simulink model "Rail_RegenerativeBraking_TianjinMetro_MotorSelection_v1"  (R2025a)
settings: Solver=ode23tb  StartTime=0.0  StopTime=SCv1.scenario.stop_time  FixedStep=Ts  MaxStep=Ts  RelTol=1e-4  EnableMultiTasking=on
PreLoadFcn:
  | SCv1_root=fileparts(fileparts(get_param(bdroot,'FileName'))); run(fullfile(SCv1_root,'config','SC_v1_parameters.m')); clear SCv1_root;
model workspace (MAT data in the model file):
  MotorCandidateIDs = {'A', 'B', 'C', 'D'}
  MotorSurrogateStatement = 'parameterized surrogate traction motor model based on published nameplate data'
  TianjinMetroBaseline.city = 'Tianjin'
  TianjinMetroBaseline.train_type = 'metro_B'
  TianjinMetroBaseline.cars = 6
  TianjinMetroBaseline.max_operation_speed_kmh = 80
  TianjinMetroBaseline.design_speed_kmh = 90
  TianjinMetroBaseline.wheel_radius_m = 0.42
  TianjinMetroBaseline.motor_count = 16
  TianjinMetroBaseline.aw2_mass_kg = 292080
  TianjinMetroBaseline.aw3_mass_kg = 316800
undefined symbols (not defined in the file): DiscIntNeverNeededParam, flux, Ld, Lq, Pn, SCv1, Ts
libraries: spsSeriesRLCBranchLib x5, spsControlledCurrentSourceLib x3, spsCurrentMeasurementLib x3, spsVoltageMeasurementLib x3, powerlib_extras x2, spsDCVoltageSourceLib x1, spsDiodeLib x1, spsPermanentMagnetSynchronousMachineLib x1, simulink x1, spsUniversalBridgeLib x1, sps_lib x1
(part 1 of 2)
Description:
  | Tianjin Metro B-type 6-car motor selection derivative. Candidate dynamics are supplied by parameterized published-nameplate FMUs.
settings Model: Creator=SUN  LastModifiedBy=AUSA
settings SolverCC: ZeroCrossControl=DisableAll  AlgebraicLoopSolver=TrustRegion
settings DataIOCC: LimitDataPoints=on  SaveFormat=Array  SignalLoggingSaveFormat=ModelDataLogs
settings OptimizationCC: ExpressionDepthLimit=2147483647.0  InitFltsAndDblsToZero=on  LifeSpan=inf
settings DebuggingCC: UnderspecifiedInitializationDetection=Classic  MergeDetectMultiDrivingBlocksExec=none  SolverPrmCheckMsg=warning  FcnCallInpInsideContextMsg=warning  UnconnectedInputMsg=warning  UnconnectedOutputMsg=warning  UnconnectedLineMsg=warning  StateNameClashWarn=warning  SFUnexpectedBacktrackingDiag=warning  SFNoUnconditionalDefaultTransitionDiag=warning  ArithmeticOperatorsInVariantConditions=warning
settings HardwareCC: ProdBitPerPointer=32.0  ProdBitPerSizeT=32.0  ProdBitPerPtrDiffT=32.0  ProdLargestAtomicFloat=None  ProdIntDivRoundTo=Undefined  ProdEndianess=Unspecified  ProdWordSize=32.0  ProdHWDeviceType=32-bit Generic
settings ModelReferenceCC: EnableRefExpFcnMdlSchedulingChecks=on  PropagateSignalLabelsOutOfModel=off
settings SFSimCC: SimUseLocalCustomCode=off  CustomCodeUndefinedFunction=UseInterfaceOnly
settings RTWCC: RTWUseLocalCustomCode=off  GPUComputeCapability=3.5
settings CodeAppCC: StateflowObjectComments=on
settings GRTTargetCC: TargetLangStandard=C89/C90 (ANSI)  CombineOutputUpdateFcns=off  GRTInterface=on
settings ConfigComp: CovMetricSettings=dw  CovSaveCumulativeToWorkspaceVar=on  CovSaveSingleToWorkspaceVar=on  CovExternalEMLEnable=off  CovSFcnEnable=off
settings SimscapeCC: SimscapeNormalizeSystem=off

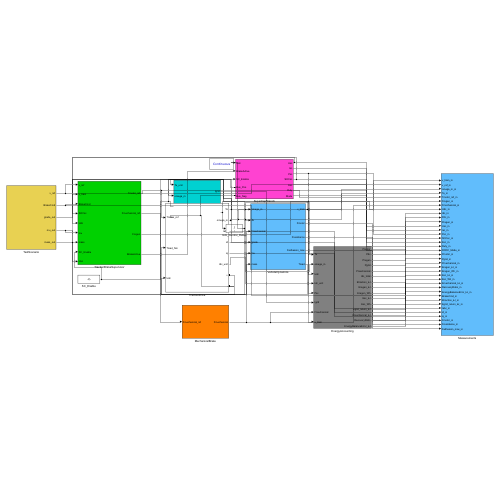
[thumbnail: Simulink's stored preview of the top-level diagram]
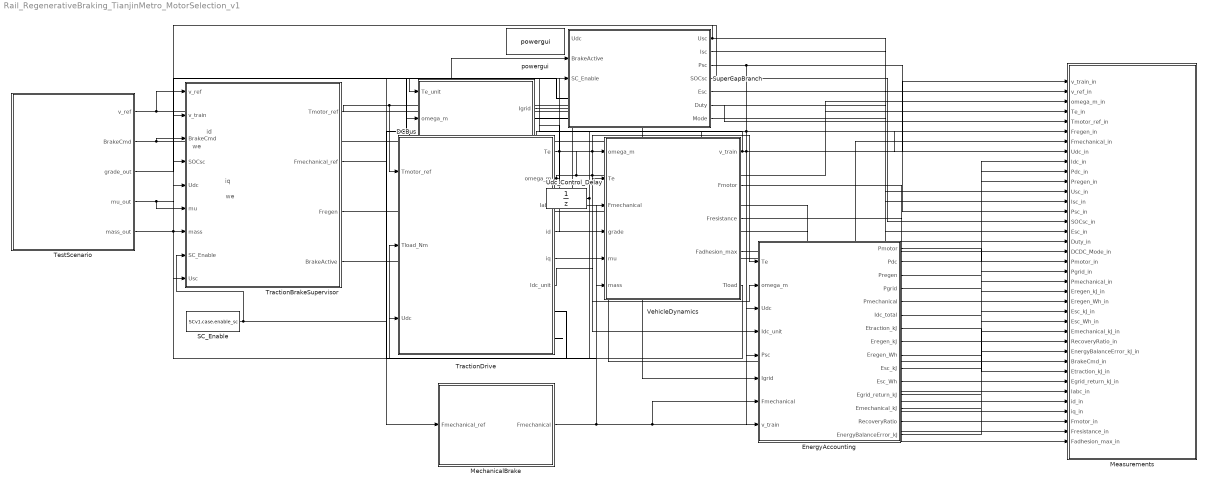
== system Rail_RegenerativeBraking_TianjinMetro_MotorSelection_v1 ==
  note: iq
  note: we
  note: we
  note: id
  DCBus : Subsystem
  EnergyAccounting : Subsystem
  Measurements : Subsystem
  MechanicalBrake : Subsystem
  SC_Enable : Constant  Value=SCv1.case.enable_sc
  SuperCapBranch : Subsystem
  TestScenario : Subsystem
  TractionBrakeSupervisor : Subsystem
  TractionDrive : Subsystem
  Udc_Control_Delay : UnitDelay  InitialCondition=SCv1.dc.Udc_initial  SampleTime=Ts  HasFrameUpgradeWarning=on
  VehicleDynamics : Subsystem
  powergui : sps_lib/powergui  SimulationMode=Continuous  SampleTime=Ts  frequency=60  Iterations=50  frequencyindice=0  Pbase=100e6  ErrMax=1e-4  UnitsV=kV  UnitsW=MW  buscounter=0  FunctionMessages=off  echomessages=off  EnableUseOfTLC=off  CurrentSourceSwitches=on  DisableSnubberDevices=off  DisableRonSwitches=off  DisableVfSwitches=off  DisplayEquations=off  AutomaticDiscreteSolvers=off  SolverType=Tustin/Backward Euler (TBE)  Interpol=off  ExternalGateDelay=off  methode=off  Ts=0  x0status=blocks  SPID=off  SwTol=0  HookPort=off  NonlinearTolerance=1e-4  nMaxIteration=100  ContinueOnMaxIteration=off  RestoreLinks=warning  ResistiveCurrentMeasurement=off  Frange=[0:2:500]  Ylog=off  Xlog=on  ShowGrid=off  save=off  variable=ZData  structure=0  ZoomFFT=on  StartTime=0.0  cycles=1  DisplayStyle=1  fundamental=60  FreqAxis=off  MaxFrequency=1000  frequencyindicesteady=1  RmsSteady=1  display=off
  wires:
  TestScenario/1(v_ref) -> TractionBrakeSupervisor/1(v_ref), Measurements/2(v_ref_in)
  VehicleDynamics/1(v_train) -> EnergyAccounting/8(v_train), Measurements/1(v_train_in), TractionBrakeSupervisor/2(v_train)
  TestScenario/2(BrakeCmd) -> TractionBrakeSupervisor/3(BrakeCmd), Measurements/29(BrakeCmd_in)
  SuperCapBranch/4(SOCsc) -> TractionBrakeSupervisor/4(SOCsc), Measurements/15(SOCsc_in)
  DCBus/2(Udc) -> EnergyAccounting/3(Udc), Measurements/8(Udc_in), Udc_Control_Delay/1
  TestScenario/4(mu_out) -> TractionBrakeSupervisor/6(mu), VehicleDynamics/5(mu)
  TestScenario/5(mass_out) -> TractionBrakeSupervisor/7(mass), VehicleDynamics/6(mass)
  SC_Enable/1 -> TractionBrakeSupervisor/8(SC_Enable), SuperCapBranch/3(SC_Enable)
  SuperCapBranch/1(Usc) -> TractionBrakeSupervisor/9(Usc), Measurements/12(Usc_in)
  TractionBrakeSupervisor/1(Tmotor_ref) -> TractionDrive/1(Tmotor_ref), Measurements/5(Tmotor_ref_in)
  TractionBrakeSupervisor/2(Fmechanical_ref) -> MechanicalBrake/1(Fmechanical_ref)
  MechanicalBrake/1(Fmechanical) -> EnergyAccounting/7(Fmechanical), Measurements/7(Fmechanical_in), VehicleDynamics/3(Fmechanical)
  TractionDrive/2(omega_m) -> EnergyAccounting/2(omega_m), Measurements/3(omega_m_in), VehicleDynamics/1(omega_m), DCBus/2(omega_m)
  TractionDrive/1(Te) -> VehicleDynamics/2(Te), EnergyAccounting/1(Te), Measurements/4(Te_in), DCBus/1(Te_unit)
  TestScenario/3(grade_out) -> VehicleDynamics/4(grade)
  VehicleDynamics/5(Tload) -> TractionDrive/2(Tload_Nm)
  TractionDrive/6(Idc_unit) -> EnergyAccounting/4(Idc_unit)
  TractionBrakeSupervisor/4(BrakeActive) -> SuperCapBranch/2(BrakeActive)
  SuperCapBranch/3(Psc) -> EnergyAccounting/5(Psc), Measurements/14(Psc_in)
  DCBus/1(Igrid) -> EnergyAccounting/6(Igrid)
  TractionBrakeSupervisor/3(Fregen) -> Measurements/6(Fregen_in)
  EnergyAccounting/6(Idc_total) -> Measurements/9(Idc_in)
  EnergyAccounting/2(Pdc) -> Measurements/10(Pdc_in)
  EnergyAccounting/3(Pregen) -> Measurements/11(Pregen_in)
  SuperCapBranch/2(Isc) -> Measurements/13(Isc_in)
  SuperCapBranch/5(Esc) -> Measurements/16(Esc_in)
  SuperCapBranch/6(Duty) -> Measurements/17(Duty_in)
  SuperCapBranch/7(Mode) -> Measurements/18(DCDC_Mode_in)
  EnergyAccounting/1(Pmotor) -> Measurements/19(Pmotor_in)
  EnergyAccounting/4(Pgrid) -> Measurements/20(Pgrid_in)
  EnergyAccounting/5(Pmechanical) -> Measurements/21(Pmechanical_in)
  EnergyAccounting/8(Eregen_kJ) -> Measurements/22(Eregen_kJ_in)
  EnergyAccounting/9(Eregen_Wh) -> Measurements/23(Eregen_Wh_in)
  EnergyAccounting/10(Esc_kJ) -> Measurements/24(Esc_kJ_in)
  EnergyAccounting/11(Esc_Wh) -> Measurements/25(Esc_Wh_in)
  EnergyAccounting/13(Emechanical_kJ) -> Measurements/26(Emechanical_kJ_in)
  EnergyAccounting/14(RecoveryRatio) -> Measurements/27(RecoveryRatio_in)
  EnergyAccounting/15(EnergyBalanceError_kJ) -> Measurements/28(EnergyBalanceError_kJ_in)
  Udc_Control_Delay/1 -> TractionDrive/3(Udc), TractionBrakeSupervisor/5(Udc), SuperCapBranch/1(Udc)
  EnergyAccounting/7(Etraction_kJ) -> Measurements/30(Etraction_kJ_in)
  EnergyAccounting/12(Egrid_return_kJ) -> Measurements/31(Egrid_return_kJ_in)
  TractionDrive/3(Iabc) -> Measurements/32(Iabc_in)
  TractionDrive/4(id) -> Measurements/33(id_in)
  TractionDrive/5(iq) -> Measurements/34(iq_in)
  VehicleDynamics/2(Fmotor) -> Measurements/35(Fmotor_in)
  VehicleDynamics/3(Fresistance) -> Measurements/36(Fresistance_in)
  VehicleDynamics/4(Fadhesion_max) -> Measurements/37(Fadhesion_max_in)
  connections:
  TractionDrive/RConn1 -- DCBus/LConn1 -- SuperCapBranch/LConn1
  TractionDrive/RConn2 -- DCBus/LConn2 -- SuperCapBranch/LConn2

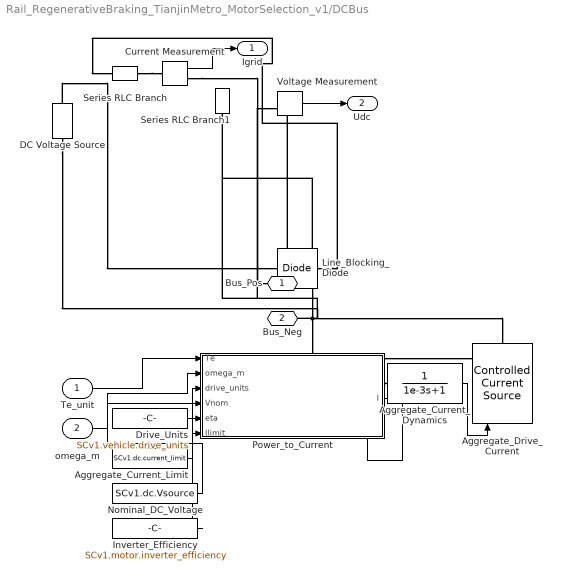
== system Rail_RegenerativeBraking_TianjinMetro_MotorSelection_v1/DCBus ==
  Te_unit : Inport
  omega_m : Inport  Port=2
  Aggregate_Current_Dynamics : TransferFcn  Numerator=1  Denominator=[1e-3 1]
  Aggregate_Current_Limit : Constant  Value=SCv1.dc.current_limit
  Aggregate_Drive_Current : spsControlledCurrentSourceLib/Controlled Current Source  Initialize=off  Source_Type=AC  Amplitude=0  Phase=0  Frequency=0  Measurements=None
  Current Measurement : spsCurrentMeasurementLib/Current Measurement  PhasorSimulation=off  OutputType=Complex  PSBequivalent=0
  DC Voltage Source : spsDCVoltageSourceLib/DC Voltage Source  Amplitude=SCv1.dc.Vsource  Measurements=None
  Drive_Units : Constant  Value=SCv1.vehicle.drive_units
  Inverter_Efficiency : Constant  Value=SCv1.motor.inverter_efficiency
  Line_Blocking_Diode : spsDiodeLib/Diode  Ron=1e-3  Lon=0  Vf=0.8  IC=0  UseSnubber=1  Rs=1e5  Cs=inf  Measurements=off
  Nominal_DC_Voltage : Constant  Value=SCv1.dc.Vsource
  Power_to_Current : MATLAB Function  TreatAsAtomicUnit=on
  Series RLC Branch : spsSeriesRLCBranchLib/Series RLC Branch  LConnTagsString=__new0  RConnTagsString=__new0  BranchType=RL  Resistance=SCv1.dc.line_R  Inductance=SCv1.dc.line_L  SetiL0=off  InitialCurrent=0  Capacitance=1e-6  Setx0=off  InitialVoltage=0  Measurements=None
  Series RLC Branch1 : spsSeriesRLCBranchLib/Series RLC Branch  LConnTagsString=__new0  RConnTagsString=__new0  BranchType=C  Resistance=25  Inductance=1e-3  SetiL0=off  InitialCurrent=0  Capacitance=SCv1.dc.Cdc  Setx0=on  InitialVoltage=SCv1.dc.Udc_initial  Measurements=None
  Voltage Measurement : spsVoltageMeasurementLib/Voltage Measurement  PhasorSimulation=off  OutputType=Complex  PSBequivalent=0
  Bus_Pos : PMIOPort  Side=Left
  Bus_Neg : PMIOPort  Port=2  Side=Left
  Igrid : Outport
  Udc : Outport  Port=2
  wires:
  Current Measurement/1 -> Igrid/1
  Voltage Measurement/1 -> Udc/1
  Power_to_Current/1(I) -> Aggregate_Current_Dynamics/1
  Aggregate_Current_Dynamics/1 -> Aggregate_Drive_Current/1
  Te_unit/1 -> Power_to_Current/1(Te)
  omega_m/1 -> Power_to_Current/2(omega_m)
  Drive_Units/1 -> Power_to_Current/3(drive_units)
  Nominal_DC_Voltage/1 -> Power_to_Current/4(Vnom)
  Inverter_Efficiency/1 -> Power_to_Current/5(eta)
  Aggregate_Current_Limit/1 -> Power_to_Current/6(Ilimit)
  connections:
  DC Voltage Source/RConn1 -- Line_Blocking_Diode/LConn1
  Line_Blocking_Diode/RConn1 -- Series RLC Branch/LConn1
  Series RLC Branch/RConn1 -- Current Measurement/LConn1
  Current Measurement/RConn1 -- Series RLC Branch1/LConn1 -- Voltage Measurement/LConn1 -- Bus_Pos/RConn1 -- Aggregate_Drive_Current/LConn1
  DC Voltage Source/LConn1 -- Series RLC Branch1/RConn1 -- Voltage Measurement/LConn2 -- Bus_Neg/RConn1 -- Aggregate_Drive_Current/RConn1

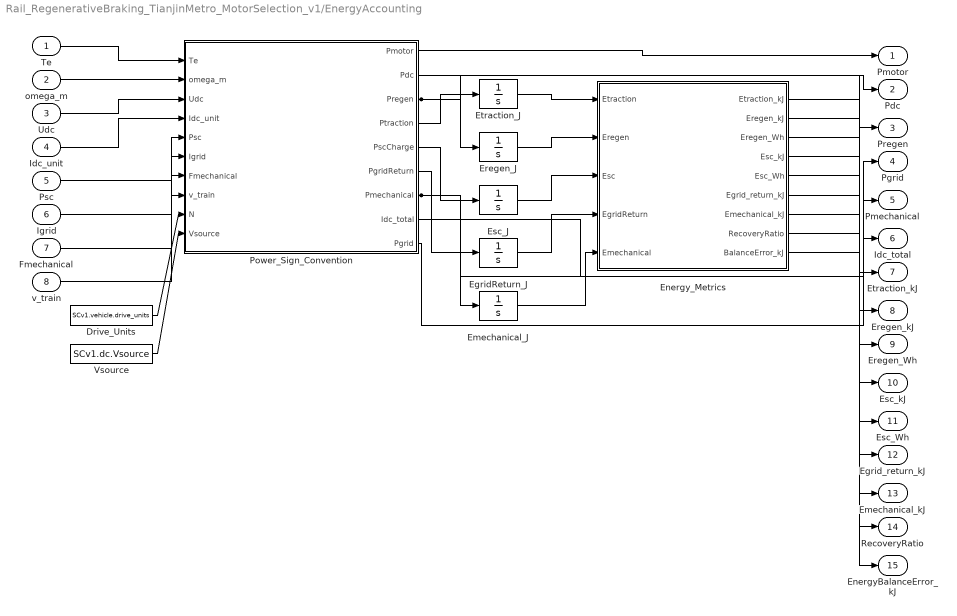
== system Rail_RegenerativeBraking_TianjinMetro_MotorSelection_v1/EnergyAccounting ==
  Te : Inport
  omega_m : Inport  Port=2
  Udc : Inport  Port=3
  Idc_unit : Inport  Port=4
  Psc : Inport  Port=5
  Igrid : Inport  Port=6
  Fmechanical : Inport  Port=7
  v_train : Inport  Port=8
  Drive_Units : Constant  Value=SCv1.vehicle.drive_units
  EgridReturn_J : Integrator
  Emechanical_J : Integrator
  Energy_Metrics : MATLAB Function  TreatAsAtomicUnit=on
  Eregen_J : Integrator
  Esc_J : Integrator
  Etraction_J : Integrator
  Power_Sign_Convention : MATLAB Function  TreatAsAtomicUnit=on
  Vsource : Constant  Value=SCv1.dc.Vsource
  Pmotor : Outport
  Pdc : Outport  Port=2
  Pregen : Outport  Port=3
  Pgrid : Outport  Port=4
  Pmechanical : Outport  Port=5
  Idc_total : Outport  Port=6
  Etraction_kJ : Outport  Port=7
  Eregen_kJ : Outport  Port=8
  Eregen_Wh : Outport  Port=9
  Esc_kJ : Outport  Port=10
  Esc_Wh : Outport  Port=11
  Egrid_return_kJ : Outport  Port=12
  Emechanical_kJ : Outport  Port=13
  RecoveryRatio : Outport  Port=14
  EnergyBalanceError_kJ : Outport  Port=15
  wires:
  Te/1 -> Power_Sign_Convention/1(Te)
  omega_m/1 -> Power_Sign_Convention/2(omega_m)
  Udc/1 -> Power_Sign_Convention/3(Udc)
  Idc_unit/1 -> Power_Sign_Convention/4(Idc_unit)
  Psc/1 -> Power_Sign_Convention/5(Psc)
  Igrid/1 -> Power_Sign_Convention/6(Igrid)
  Fmechanical/1 -> Power_Sign_Convention/7(Fmechanical)
  v_train/1 -> Power_Sign_Convention/8(v_train)
  Drive_Units/1 -> Power_Sign_Convention/9(N)
  Vsource/1 -> Power_Sign_Convention/10(Vsource)
  Power_Sign_Convention/4(Ptraction) -> Etraction_J/1
  Power_Sign_Convention/3(Pregen) -> Eregen_J/1, Pregen/1
  Power_Sign_Convention/5(PscCharge) -> Esc_J/1
  Power_Sign_Convention/6(PgridReturn) -> EgridReturn_J/1
  Power_Sign_Convention/7(Pmechanical) -> Emechanical_J/1, Pmechanical/1
  Etraction_J/1 -> Energy_Metrics/1(Etraction)
  Eregen_J/1 -> Energy_Metrics/2(Eregen)
  Esc_J/1 -> Energy_Metrics/3(Esc)
  EgridReturn_J/1 -> Energy_Metrics/4(EgridReturn)
  Emechanical_J/1 -> Energy_Metrics/5(Emechanical)
  Power_Sign_Convention/1(Pmotor) -> Pmotor/1
  Power_Sign_Convention/2(Pdc) -> Pdc/1
  Power_Sign_Convention/9(Pgrid) -> Pgrid/1
  Power_Sign_Convention/8(Idc_total) -> Idc_total/1
  Energy_Metrics/1(Etraction_kJ) -> Etraction_kJ/1
  Energy_Metrics/2(Eregen_kJ) -> Eregen_kJ/1
  Energy_Metrics/3(Eregen_Wh) -> Eregen_Wh/1
  Energy_Metrics/4(Esc_kJ) -> Esc_kJ/1
  Energy_Metrics/5(Esc_Wh) -> Esc_Wh/1
  Energy_Metrics/6(Egrid_return_kJ) -> Egrid_return_kJ/1
  Energy_Metrics/7(Emechanical_kJ) -> Emechanical_kJ/1
  Energy_Metrics/8(RecoveryRatio) -> RecoveryRatio/1
  Energy_Metrics/9(BalanceError_kJ) -> EnergyBalanceError_kJ/1

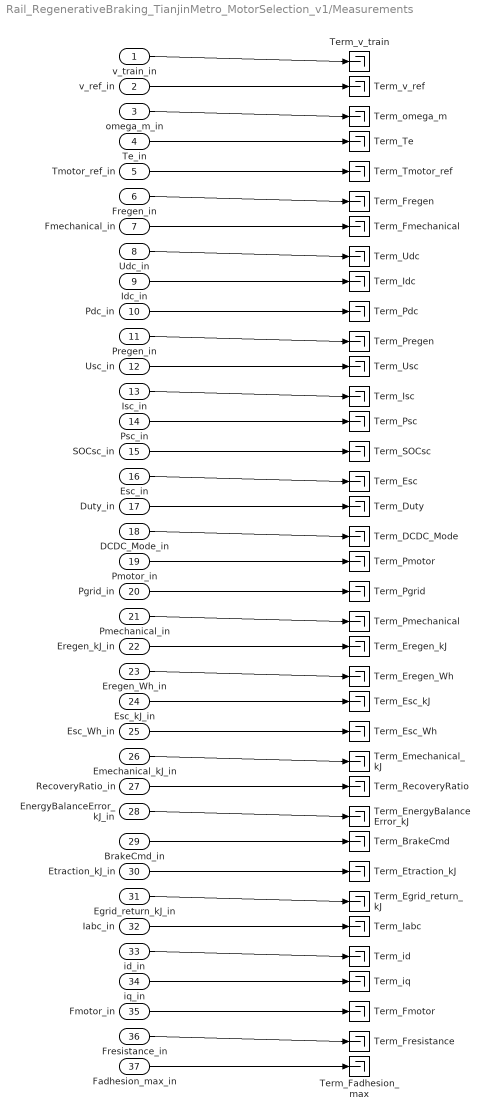
== system Rail_RegenerativeBraking_TianjinMetro_MotorSelection_v1/Measurements ==
  v_train_in : Inport
  v_ref_in : Inport  Port=2
  omega_m_in : Inport  Port=3
  Te_in : Inport  Port=4
  Tmotor_ref_in : Inport  Port=5
  Fregen_in : Inport  Port=6
  Fmechanical_in : Inport  Port=7
  Udc_in : Inport  Port=8
  Idc_in : Inport  Port=9
  Pdc_in : Inport  Port=10
  Pregen_in : Inport  Port=11
  Usc_in : Inport  Port=12
  Isc_in : Inport  Port=13
  Psc_in : Inport  Port=14
  SOCsc_in : Inport  Port=15
  Esc_in : Inport  Port=16
  Duty_in : Inport  Port=17
  DCDC_Mode_in : Inport  Port=18
  Pmotor_in : Inport  Port=19
  Pgrid_in : Inport  Port=20
  Pmechanical_in : Inport  Port=21
  Eregen_kJ_in : Inport  Port=22
  Eregen_Wh_in : Inport  Port=23
  Esc_kJ_in : Inport  Port=24
  Esc_Wh_in : Inport  Port=25
  Emechanical_kJ_in : Inport  Port=26
  RecoveryRatio_in : Inport  Port=27
  EnergyBalanceError_kJ_in : Inport  Port=28
  BrakeCmd_in : Inport  Port=29
  Etraction_kJ_in : Inport  Port=30
  Egrid_return_kJ_in : Inport  Port=31
  Iabc_in : Inport  Port=32
  id_in : Inport  Port=33
  iq_in : Inport  Port=34
  Fmotor_in : Inport  Port=35
  Fresistance_in : Inport  Port=36
  Fadhesion_max_in : Inport  Port=37
  Term_BrakeCmd : Terminator
  Term_DCDC_Mode : Terminator
  Term_Duty : Terminator
  Term_Egrid_return_kJ : Terminator
  Term_Emechanical_kJ : Terminator
  Term_EnergyBalanceError_kJ : Terminator
  Term_Eregen_Wh : Terminator
  Term_Eregen_kJ : Terminator
  Term_Esc : Terminator
  Term_Esc_Wh : Terminator
  Term_Esc_kJ : Terminator
  Term_Etraction_kJ : Terminator
  Term_Fadhesion_max : Terminator
  Term_Fmechanical : Terminator
  Term_Fmotor : Terminator
  Term_Fregen : Terminator
  Term_Fresistance : Terminator
  Term_Iabc : Terminator
  Term_Idc : Terminator
  Term_Isc : Terminator
  Term_Pdc : Terminator
  Term_Pgrid : Terminator
  Term_Pmechanical : Terminator
  Term_Pmotor : Terminator
  Term_Pregen : Terminator
  Term_Psc : Terminator
  Term_RecoveryRatio : Terminator
  Term_SOCsc : Terminator
  Term_Te : Terminator
  Term_Tmotor_ref : Terminator
  Term_Udc : Terminator
  Term_Usc : Terminator
  Term_id : Terminator
  Term_iq : Terminator
  Term_omega_m : Terminator
  Term_v_ref : Terminator
  Term_v_train : Terminator
  wires:
  v_train_in/1 -> Term_v_train/1
  v_ref_in/1 -> Term_v_ref/1
  omega_m_in/1 -> Term_omega_m/1
  Te_in/1 -> Term_Te/1
  Tmotor_ref_in/1 -> Term_Tmotor_ref/1
  Fregen_in/1 -> Term_Fregen/1
  Fmechanical_in/1 -> Term_Fmechanical/1
  Udc_in/1 -> Term_Udc/1
  Idc_in/1 -> Term_Idc/1
  Pdc_in/1 -> Term_Pdc/1
  Pregen_in/1 -> Term_Pregen/1
  Usc_in/1 -> Term_Usc/1
  Isc_in/1 -> Term_Isc/1
  Psc_in/1 -> Term_Psc/1
  SOCsc_in/1 -> Term_SOCsc/1
  Esc_in/1 -> Term_Esc/1
  Duty_in/1 -> Term_Duty/1
  DCDC_Mode_in/1 -> Term_DCDC_Mode/1
  Pmotor_in/1 -> Term_Pmotor/1
  Pgrid_in/1 -> Term_Pgrid/1
  Pmechanical_in/1 -> Term_Pmechanical/1
  Eregen_kJ_in/1 -> Term_Eregen_kJ/1
  Eregen_Wh_in/1 -> Term_Eregen_Wh/1
  Esc_kJ_in/1 -> Term_Esc_kJ/1
  Esc_Wh_in/1 -> Term_Esc_Wh/1
  Emechanical_kJ_in/1 -> Term_Emechanical_kJ/1
  RecoveryRatio_in/1 -> Term_RecoveryRatio/1
  EnergyBalanceError_kJ_in/1 -> Term_EnergyBalanceError_kJ/1
  BrakeCmd_in/1 -> Term_BrakeCmd/1
  Etraction_kJ_in/1 -> Term_Etraction_kJ/1
  Egrid_return_kJ_in/1 -> Term_Egrid_return_kJ/1
  Iabc_in/1 -> Term_Iabc/1
  id_in/1 -> Term_id/1
  iq_in/1 -> Term_iq/1
  Fmotor_in/1 -> Term_Fmotor/1
  Fresistance_in/1 -> Term_Fresistance/1
  Fadhesion_max_in/1 -> Term_Fadhesion_max/1

== system Rail_RegenerativeBraking_TianjinMetro_MotorSelection_v1/MechanicalBrake ==
  Fmechanical_ref : Inport
  Brake_Lag : TransferFcn  Numerator=1  Denominator=[SCv1.brake.mechanical_tau 1]
  Force_Limit : Saturate  UpperLimit=SCv1.brake.mechanical_force_max  LowerLimit=0
  Fmechanical : Outport
  wires:
  Fmechanical_ref/1 -> Force_Limit/1
  Force_Limit/1 -> Brake_Lag/1
  Brake_Lag/1 -> Fmechanical/1

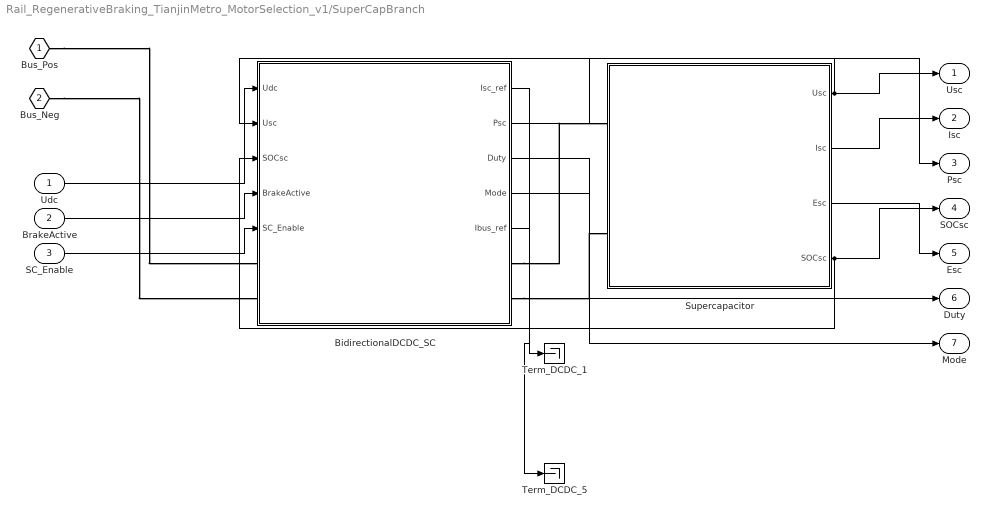
== system Rail_RegenerativeBraking_TianjinMetro_MotorSelection_v1/SuperCapBranch ==
  Udc : Inport
  BrakeActive : Inport  Port=2
  SC_Enable : Inport  Port=3
  BidirectionalDCDC_SC : Subsystem
  Supercapacitor : Subsystem
  Term_DCDC_1 : Terminator
  Term_DCDC_5 : Terminator
  Bus_Pos : PMIOPort  Side=Left
  Bus_Neg : PMIOPort  Port=2  Side=Left
  Usc : Outport
  Isc : Outport  Port=2
  Psc : Outport  Port=3
  SOCsc : Outport  Port=4
  Esc : Outport  Port=5
  Duty : Outport  Port=6
  Mode : Outport  Port=7
  wires:
  Udc/1 -> BidirectionalDCDC_SC/1(Udc)
  Supercapacitor/1(Usc) -> BidirectionalDCDC_SC/2(Usc), Usc/1
  Supercapacitor/4(SOCsc) -> BidirectionalDCDC_SC/3(SOCsc), SOCsc/1
  BrakeActive/1 -> BidirectionalDCDC_SC/4(BrakeActive)
  SC_Enable/1 -> BidirectionalDCDC_SC/5(SC_Enable)
  Supercapacitor/2(Isc) -> Isc/1
  BidirectionalDCDC_SC/2(Psc) -> Psc/1
  Supercapacitor/3(Esc) -> Esc/1
  BidirectionalDCDC_SC/3(Duty) -> Duty/1
  BidirectionalDCDC_SC/4(Mode) -> Mode/1
  BidirectionalDCDC_SC/1(Isc_ref) -> Term_DCDC_1/1
  BidirectionalDCDC_SC/5(Ibus_ref) -> Term_DCDC_5/1
  connections:
  Bus_Pos/RConn1 -- BidirectionalDCDC_SC/LConn1
  Bus_Neg/RConn1 -- BidirectionalDCDC_SC/LConn2
  BidirectionalDCDC_SC/RConn1 -- Supercapacitor/LConn1
  BidirectionalDCDC_SC/RConn2 -- Supercapacitor/LConn2

== system Rail_RegenerativeBraking_TianjinMetro_MotorSelection_v1/TestScenario ==
  Clock : Clock
  Speed_Profile : MATLAB Function  TreatAsAtomicUnit=on
  accel : Constant  Value=SCv1.scenario.acceleration
  brake_start : Constant  Value=SCv1.scenario.brake_start
  decel : Constant  Value=SCv1.brake.deceleration
  grade : Constant  Value=SCv1.vehicle.grade
  mass : Constant  Value=SCv1.vehicle.mass
  mu : Constant  Value=SCv1.vehicle.mu
  start_time : Constant  Value=SCv1.scenario.start_time
  target_speed : Constant  Value=SCv1.scenario.target_speed
  v_ref : Outport
  BrakeCmd : Outport  Port=2
  grade_out : Outport  Port=3
  mu_out : Outport  Port=4
  mass_out : Outport  Port=5
  wires:
  Clock/1 -> Speed_Profile/1(t)
  target_speed/1 -> Speed_Profile/2(target_speed)
  accel/1 -> Speed_Profile/3(accel)
  start_time/1 -> Speed_Profile/4(start_time)
  brake_start/1 -> Speed_Profile/5(brake_start)
  decel/1 -> Speed_Profile/6(decel)
  Speed_Profile/1(v_ref) -> v_ref/1
  Speed_Profile/2(BrakeCmd) -> BrakeCmd/1
  grade/1 -> grade_out/1
  mu/1 -> mu_out/1
  mass/1 -> mass_out/1

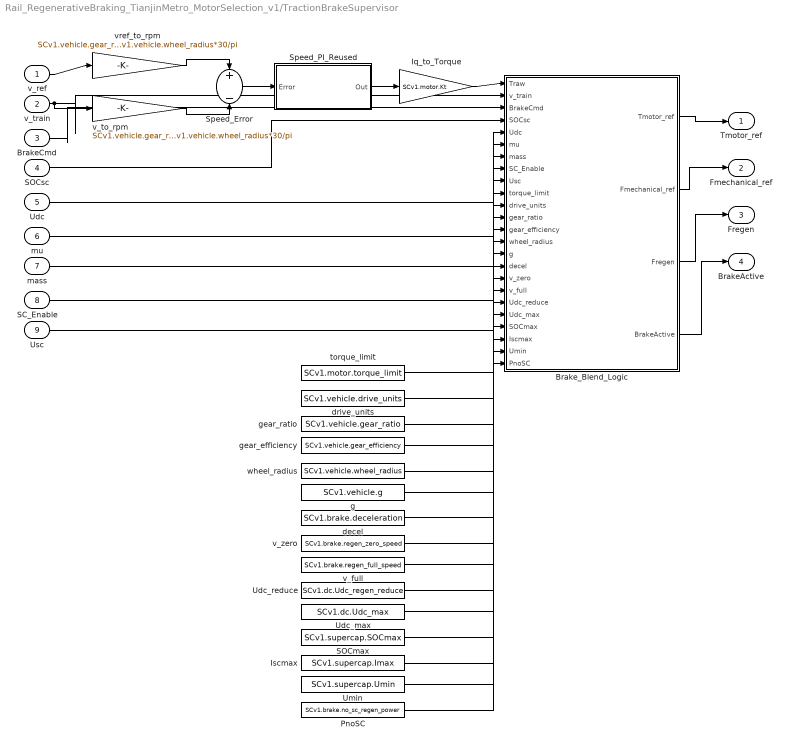
== system Rail_RegenerativeBraking_TianjinMetro_MotorSelection_v1/TractionBrakeSupervisor ==
  v_ref : Inport
  v_train : Inport  Port=2
  BrakeCmd : Inport  Port=3
  SOCsc : Inport  Port=4
  Udc : Inport  Port=5
  mu : Inport  Port=6
  mass : Inport  Port=7
  SC_Enable : Inport  Port=8
  Usc : Inport  Port=9
  Brake_Blend_Logic : MATLAB Function  TreatAsAtomicUnit=on
  Iq_to_Torque : Gain  Gain=SCv1.motor.Kt
  Iscmax : Constant  Value=SCv1.supercap.Imax
  PnoSC : Constant  Value=SCv1.brake.no_sc_regen_power
  SOCmax : Constant  Value=SCv1.supercap.SOCmax
  Speed_Error : Sum  Inputs=+-
  Speed_PI_Reused : Subsystem  AncestorBlock=|  DialogController=POWERSYS.PowerSysDialog  mask(Discrete PI Controller){Kpw=2.595, Kiw=40.94, Ba=0.013, Par_Limits=[180 -180], Init=0, Ts=Ts}
      | powerlib_extras/Discrete 
      | Control Blocks/Discrete
      | PI Controller
      mask prompts: Kpw "Proportional gain (Kp):"; Kiw "Integral gain (Ki):"; Ba "feedback gain (Ba)"; Par_Limits "Output limits: [ Upper   Lower ]"; Init "Output initial value:"; Ts "Sample time:"
      mask help: This block implements a discrete PI controller.
      mask init:
      | UpperLimit=Par_Limits(1);
      | LowerLimit=Par_Limits(2);
      | power_initmask();
      mask Help: This block is part of a subset of blocks in the Extras library that does not have documentation associated with it, other than the block mask description.
      mask Display: disp('PI');
  Udc_max : Constant  Value=SCv1.dc.Udc_max
  Udc_reduce : Constant  Value=SCv1.dc.Udc_regen_reduce
  Umin : Constant  Value=SCv1.supercap.Umin
  decel : Constant  Value=SCv1.brake.deceleration
  drive_units : Constant  Value=SCv1.vehicle.drive_units
  g : Constant  Value=SCv1.vehicle.g
  gear_efficiency : Constant  Value=SCv1.vehicle.gear_efficiency
  gear_ratio : Constant  Value=SCv1.vehicle.gear_ratio
  torque_limit : Constant  Value=SCv1.motor.torque_limit
  v_full : Constant  Value=SCv1.brake.regen_full_speed
  v_to_rpm : Gain  Gain=SCv1.vehicle.gear_ratio/SCv1.vehicle.wheel_radius*30/pi
  v_zero : Constant  Value=SCv1.brake.regen_zero_speed
  vref_to_rpm : Gain  Gain=SCv1.vehicle.gear_ratio/SCv1.vehicle.wheel_radius*30/pi
  wheel_radius : Constant  Value=SCv1.vehicle.wheel_radius
  Tmotor_ref : Outport
  Fmechanical_ref : Outport  Port=2
  Fregen : Outport  Port=3
  BrakeActive : Outport  Port=4
  wires:
  v_ref/1 -> vref_to_rpm/1
  vref_to_rpm/1 -> Speed_Error/1
  v_train/1 -> v_to_rpm/1, Brake_Blend_Logic/2(v_train)
  v_to_rpm/1 -> Speed_Error/2
  Speed_Error/1 -> Speed_PI_Reused/1(Error)
  Speed_PI_Reused/1(Out) -> Iq_to_Torque/1
  Iq_to_Torque/1 -> Brake_Blend_Logic/1(Traw)
  BrakeCmd/1 -> Brake_Blend_Logic/3(BrakeCmd)
  SOCsc/1 -> Brake_Blend_Logic/4(SOCsc)
  Udc/1 -> Brake_Blend_Logic/5(Udc)
  mu/1 -> Brake_Blend_Logic/6(mu)
  mass/1 -> Brake_Blend_Logic/7(mass)
  SC_Enable/1 -> Brake_Blend_Logic/8(SC_Enable)
  Usc/1 -> Brake_Blend_Logic/9(Usc)
  torque_limit/1 -> Brake_Blend_Logic/10(torque_limit)
  drive_units/1 -> Brake_Blend_Logic/11(drive_units)
  gear_ratio/1 -> Brake_Blend_Logic/12(gear_ratio)
  gear_efficiency/1 -> Brake_Blend_Logic/13(gear_efficiency)
  wheel_radius/1 -> Brake_Blend_Logic/14(wheel_radius)
  g/1 -> Brake_Blend_Logic/15(g)
  decel/1 -> Brake_Blend_Logic/16(decel)
  v_zero/1 -> Brake_Blend_Logic/17(v_zero)
  v_full/1 -> Brake_Blend_Logic/18(v_full)
  Udc_reduce/1 -> Brake_Blend_Logic/19(Udc_reduce)
  Udc_max/1 -> Brake_Blend_Logic/20(Udc_max)
  SOCmax/1 -> Brake_Blend_Logic/21(SOCmax)
  Iscmax/1 -> Brake_Blend_Logic/22(Iscmax)
  Umin/1 -> Brake_Blend_Logic/23(Umin)
  PnoSC/1 -> Brake_Blend_Logic/24(PnoSC)
  Brake_Blend_Logic/1(Tmotor_ref) -> Tmotor_ref/1
  Brake_Blend_Logic/2(Fmechanical_ref) -> Fmechanical_ref/1
  Brake_Blend_Logic/3(Fregen) -> Fregen/1
  Brake_Blend_Logic/4(BrakeActive) -> BrakeActive/1

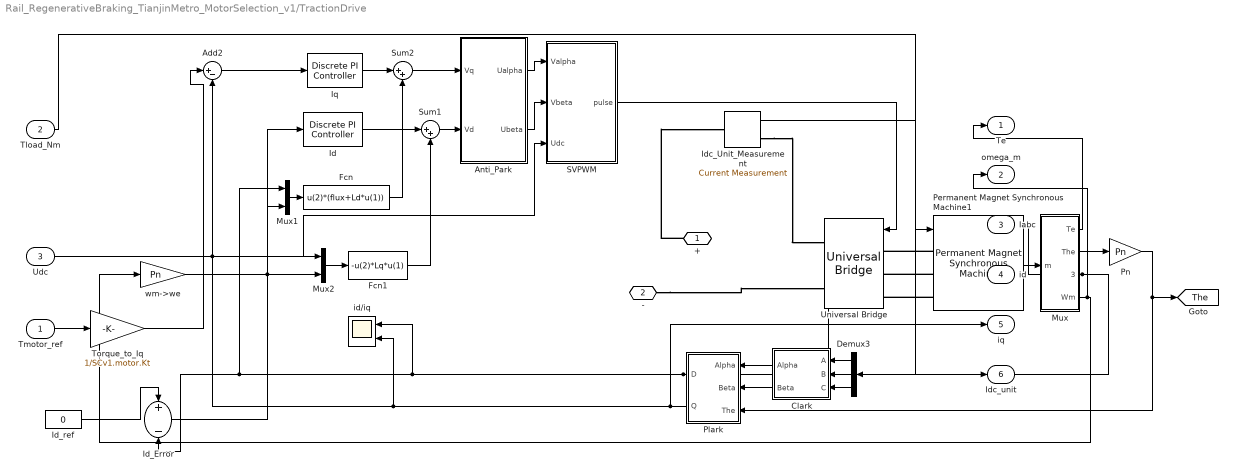
== system Rail_RegenerativeBraking_TianjinMetro_MotorSelection_v1/TractionDrive ==
  Tmotor_ref : Inport
  Tload_Nm : Inport  Port=2
  Udc : Inport  Port=3
  Add2 : Sum  Inputs=|+-
  Anti_Park : Subsystem
  Clark : Subsystem
  Demux3 : Demux  Outputs=3
  Fcn : Fcn  Expr=u(2)*(flux+Ld*u(1))
  Fcn1 : Fcn  Expr=-u(2)*Lq*u(1)
  Id : powerlib_extras/Discrete  Control Blocks/Discrete PI Controller  Kp=25.7  Ki=300  Par_Limits=[1500*0.9*sqrt(1/3) -1500*0.9*sqrt(1/3)]  Init=0  Ts=Ts
  Id_Error : Sum  Inputs=+-
  Id_ref : Constant  Value=0
  Idc_Unit_Measurement : spsCurrentMeasurementLib/Current Measurement  PhasorSimulation=off  OutputType=Complex  PSBequivalent=0
  Iq : powerlib_extras/Discrete  Control Blocks/Discrete PI Controller  Kp=25.7  Ki=300  Par_Limits=[1500*0.9*sqrt(1/3) -1500*0.9*sqrt(1/3)]  Init=0  Ts=Ts
  Mux : Subsystem
  Mux1 : Mux  Inputs=2
  Mux2 : Mux  Inputs=2
  Permanent Magnet Synchronous Machine1 : spsPermanentMagnetSynchronousMachineLib/Permanent Magnet Synchronous Machine  NbPhases=3  FluxDistribution=Sinusoidal  RotorType=Salient-pole  MechanicalLoad=Torque Tm  PresetModel=No  ShowDetailedParameters=on  MeasurementBus=off  Resistance=0.285  Inductance=8.5e-3  dqInductances=[2.5e-3,2.5e-3]  La=0.000835  MachineConstant=Flux linkage established by magnets (V.s)  Flux=0.75  VoltageCst=544.1398  TorqueCst=4.5  Flat=120  Mechanical=[SCv1.motor.J_equivalent SCv1.motor.B_motor 4]  PolePairs=3  InitialConditions=[0,0, 0,0]  InitialConditions5ph=[0 0 0 0 0 0]  RefAngle=Aligned with phase A axis (original Park)  IterativeDiscreteModel=Trapezoidal non iterative  TsBlock=-1  TsPowergui=0
  Plark : Subsystem
  Pn : Gain  Gain=Pn
  SVPWM : Subsystem
  Sum1 : Sum  Inputs=|++
  Sum2 : Sum  Inputs=|++
  Torque_to_Iq : Gain  Gain=1/SCv1.motor.Kt
  Universal Bridge : spsUniversalBridgeLib/Universal Bridge  Arms=3  SnubberResistance=1e5  SnubberCapacitance=inf  Device=IGBT / Diodes  Ron=1e-3  Lon=0  ForwardVoltages="[  0  0  ]"  ForwardVoltage=0  GTOparameters=[ 10e-6 , 20e-6 ]  IGBTparameters=[ 1e-6 , 2e-6 ]  Measurements=None  Measurements_2=None  converterType=Rectifier
  id/iq : Scope  NumInputPorts=2
      settings: ActiveDisplayYMinimum=-181.97295  ActiveDisplayYMaximum=204.25765
  wm->we : Gain  Gain=Pn
  + : PMIOPort  Side=Right
  - : PMIOPort  Port=2  Side=Right
  Te : Outport
  omega_m : Outport  Port=2
  Iabc : Outport  Port=3
  id : Outport  Port=4
  iq : Outport  Port=5
  Idc_unit : Outport  Port=6
  tag scope: The=global
  wires:
  Id/1 -> Sum1/1
  Fcn1/1 -> Sum1/2
  SVPWM/1(pulse) -> Universal Bridge/1
  Fcn/1 -> Sum2/2
  wm->we/1 -> Mux2/2, Mux1/2
  Plark/2(Q) -> id/iq/2, Mux2/1, Add2/2, iq/1
  Plark/1(D) -> Id_Error/2, Mux1/1, id/iq/1, id/1
  Mux/2(The) -> Pn/1
  Sum2/1 -> Anti_Park/1(Vq)
  Mux1/1 -> Fcn/1
  Mux/4(Wm) -> omega_m/1, wm->we/1
  Pn/1 -> Plark/3(The), [The]
  Permanent Magnet Synchronous Machine1/1 -> Mux/1(m)
  Mux2/1 -> Fcn1/1
  Clark/1(Alpha) -> Plark/1(Alpha)
  Iq/1 -> Sum2/1
  Mux/3(Iabc) -> Iabc/1, Demux3/1
  Anti_Park/1(Ualpha) -> SVPWM/1(Valpha)
  Clark/2(Beta) -> Plark/2(Beta)
  Demux3/1 -> Clark/1(A)
  Demux3/3 -> Clark/3(C)
  Add2/1 -> Iq/1
  Sum1/1 -> Anti_Park/2(Vd)
  Demux3/2 -> Clark/2(B)
  Anti_Park/2(Ubeta) -> SVPWM/2(Vbeta)
  Mux/1(Te) -> Te/1
  Id_ref/1 -> Id_Error/1
  Id_Error/1 -> Id/1
  Tmotor_ref/1 -> Torque_to_Iq/1
  Torque_to_Iq/1 -> Add2/1
  Tload_Nm/1 -> Permanent Magnet Synchronous Machine1/1
  Udc/1 -> SVPWM/3(Udc)
  Idc_Unit_Measurement/1 -> Idc_unit/1
  connections:
  Permanent Magnet Synchronous Machine1/LConn2 -- Universal Bridge/LConn2
  Permanent Magnet Synchronous Machine1/LConn3 -- Universal Bridge/LConn3
  -/RConn1 -- Universal Bridge/RConn2
  Permanent Magnet Synchronous Machine1/LConn1 -- Universal Bridge/LConn1
  +/RConn1 -- Idc_Unit_Measurement/LConn1
  Idc_Unit_Measurement/RConn1 -- Universal Bridge/RConn1

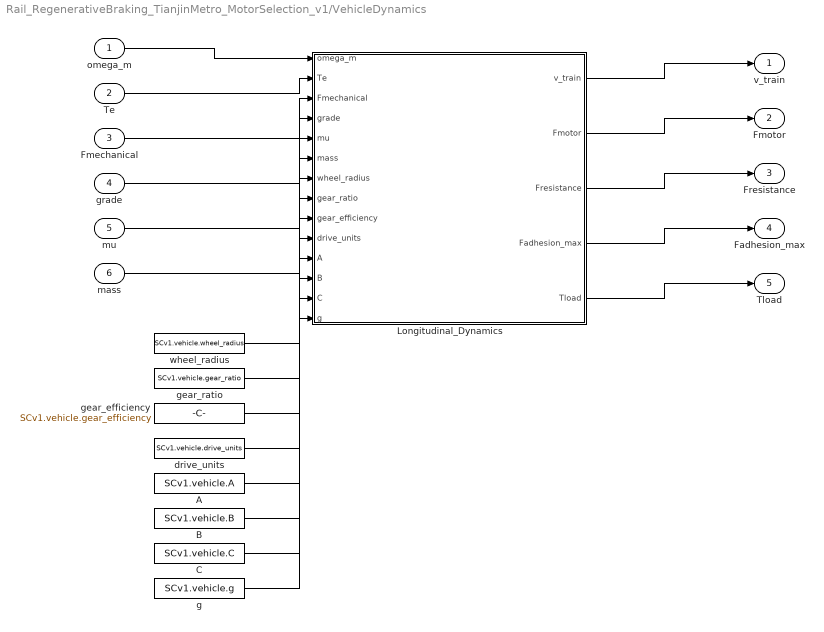
== system Rail_RegenerativeBraking_TianjinMetro_MotorSelection_v1/VehicleDynamics ==
  omega_m : Inport
  Te : Inport  Port=2
  Fmechanical : Inport  Port=3
  grade : Inport  Port=4
  mu : Inport  Port=5
  mass : Inport  Port=6
  A : Constant  Value=SCv1.vehicle.A
  B : Constant  Value=SCv1.vehicle.B
  C : Constant  Value=SCv1.vehicle.C
  Longitudinal_Dynamics : MATLAB Function  TreatAsAtomicUnit=on
  drive_units : Constant  Value=SCv1.vehicle.drive_units
  g : Constant  Value=SCv1.vehicle.g
  gear_efficiency : Constant  Value=SCv1.vehicle.gear_efficiency
  gear_ratio : Constant  Value=SCv1.vehicle.gear_ratio
  wheel_radius : Constant  Value=SCv1.vehicle.wheel_radius
  v_train : Outport
  Fmotor : Outport  Port=2
  Fresistance : Outport  Port=3
  Fadhesion_max : Outport  Port=4
  Tload : Outport  Port=5
  wires:
  omega_m/1 -> Longitudinal_Dynamics/1(omega_m)
  Te/1 -> Longitudinal_Dynamics/2(Te)
  Fmechanical/1 -> Longitudinal_Dynamics/3(Fmechanical)
  grade/1 -> Longitudinal_Dynamics/4(grade)
  mu/1 -> Longitudinal_Dynamics/5(mu)
  mass/1 -> Longitudinal_Dynamics/6(mass)
  wheel_radius/1 -> Longitudinal_Dynamics/7(wheel_radius)
  gear_ratio/1 -> Longitudinal_Dynamics/8(gear_ratio)
  gear_efficiency/1 -> Longitudinal_Dynamics/9(gear_efficiency)
  drive_units/1 -> Longitudinal_Dynamics/10(drive_units)
  A/1 -> Longitudinal_Dynamics/11(A)
  B/1 -> Longitudinal_Dynamics/12(B)
  C/1 -> Longitudinal_Dynamics/13(C)
  g/1 -> Longitudinal_Dynamics/14(g)
  Longitudinal_Dynamics/1(v_train) -> v_train/1
  Longitudinal_Dynamics/2(Fmotor) -> Fmotor/1
  Longitudinal_Dynamics/3(Fresistance) -> Fresistance/1
  Longitudinal_Dynamics/4(Fadhesion_max) -> Fadhesion_max/1
  Longitudinal_Dynamics/5(Tload) -> Tload/1

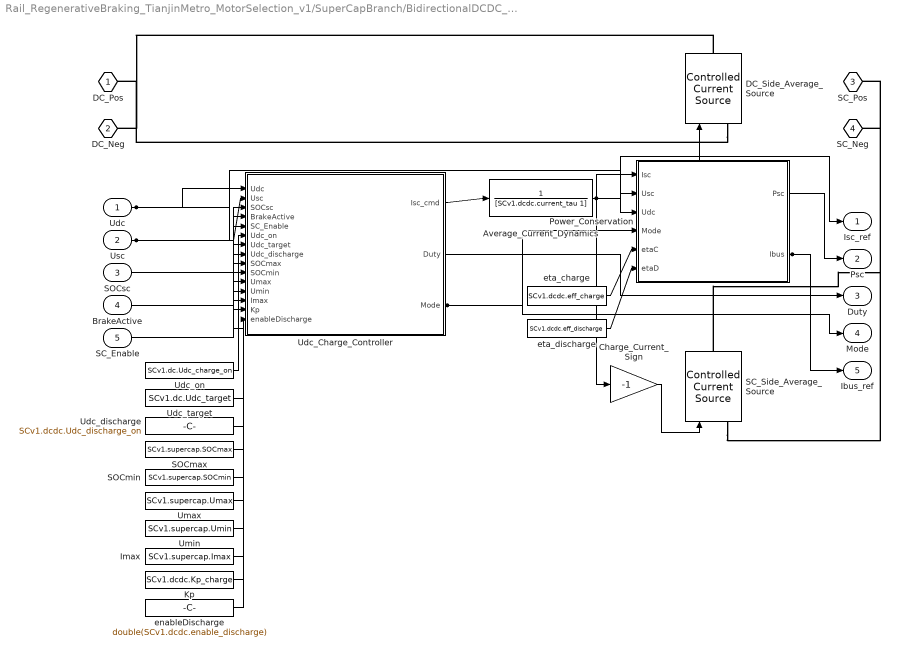
== system Rail_RegenerativeBraking_TianjinMetro_MotorSelection_v1/SuperCapBranch/BidirectionalDCDC_SC ==
  Udc : Inport
  Usc : Inport  Port=2
  SOCsc : Inport  Port=3
  BrakeActive : Inport  Port=4
  SC_Enable : Inport  Port=5
  Average_Current_Dynamics : TransferFcn  Numerator=1  Denominator=[SCv1.dcdc.current_tau 1]
  Charge_Current_Sign : Gain  Gain=-1
  DC_Side_Average_Source : spsControlledCurrentSourceLib/Controlled Current Source  Initialize=off  Source_Type=AC  Amplitude=0  Phase=0  Frequency=0  Measurements=None
  Imax : Constant  Value=SCv1.supercap.Imax
  Kp : Constant  Value=SCv1.dcdc.Kp_charge
  Power_Conservation : MATLAB Function  TreatAsAtomicUnit=on
  SC_Side_Average_Source : spsControlledCurrentSourceLib/Controlled Current Source  Initialize=off  Source_Type=AC  Amplitude=0  Phase=0  Frequency=0  Measurements=None
  SOCmax : Constant  Value=SCv1.supercap.SOCmax
  SOCmin : Constant  Value=SCv1.supercap.SOCmin
  Udc_Charge_Controller : MATLAB Function  TreatAsAtomicUnit=on
  Udc_discharge : Constant  Value=SCv1.dcdc.Udc_discharge_on
  Udc_on : Constant  Value=SCv1.dc.Udc_charge_on
  Udc_target : Constant  Value=SCv1.dc.Udc_target
  Umax : Constant  Value=SCv1.supercap.Umax
  Umin : Constant  Value=SCv1.supercap.Umin
  enableDischarge : Constant  Value=double(SCv1.dcdc.enable_discharge)
  eta_charge : Constant  Value=SCv1.dcdc.eff_charge
  eta_discharge : Constant  Value=SCv1.dcdc.eff_discharge
  DC_Pos : PMIOPort  Side=Left
  DC_Neg : PMIOPort  Port=2  Side=Left
  SC_Pos : PMIOPort  Port=3  Side=Right
  SC_Neg : PMIOPort  Port=4  Side=Right
  Isc_ref : Outport
  Psc : Outport  Port=2
  Duty : Outport  Port=3
  Mode : Outport  Port=4
  Ibus_ref : Outport  Port=5
  wires:
  Udc/1 -> Udc_Charge_Controller/1(Udc), Power_Conservation/3(Udc)
  Usc/1 -> Udc_Charge_Controller/2(Usc), Power_Conservation/2(Usc)
  SOCsc/1 -> Udc_Charge_Controller/3(SOCsc)
  BrakeActive/1 -> Udc_Charge_Controller/4(BrakeActive)
  SC_Enable/1 -> Udc_Charge_Controller/5(SC_Enable)
  Udc_on/1 -> Udc_Charge_Controller/6(Udc_on)
  Udc_target/1 -> Udc_Charge_Controller/7(Udc_target)
  Udc_discharge/1 -> Udc_Charge_Controller/8(Udc_discharge)
  SOCmax/1 -> Udc_Charge_Controller/9(SOCmax)
  SOCmin/1 -> Udc_Charge_Controller/10(SOCmin)
  Umax/1 -> Udc_Charge_Controller/11(Umax)
  Umin/1 -> Udc_Charge_Controller/12(Umin)
  Imax/1 -> Udc_Charge_Controller/13(Imax)
  Kp/1 -> Udc_Charge_Controller/14(Kp)
  enableDischarge/1 -> Udc_Charge_Controller/15(enableDischarge)
  Udc_Charge_Controller/1(Isc_cmd) -> Average_Current_Dynamics/1
  Average_Current_Dynamics/1 -> Power_Conservation/1(Isc), Charge_Current_Sign/1, Isc_ref/1
  Udc_Charge_Controller/3(Mode) -> Power_Conservation/4(Mode), Mode/1
  eta_charge/1 -> Power_Conservation/5(etaC)
  eta_discharge/1 -> Power_Conservation/6(etaD)
  Power_Conservation/2(Ibus) -> DC_Side_Average_Source/1, Ibus_ref/1
  Charge_Current_Sign/1 -> SC_Side_Average_Source/1
  Power_Conservation/1(Psc) -> Psc/1
  Udc_Charge_Controller/2(Duty) -> Duty/1
  connections:
  DC_Side_Average_Source/LConn1 -- DC_Pos/RConn1
  DC_Side_Average_Source/RConn1 -- DC_Neg/RConn1
  SC_Side_Average_Source/LConn1 -- SC_Pos/RConn1
  SC_Side_Average_Source/RConn1 -- SC_Neg/RConn1

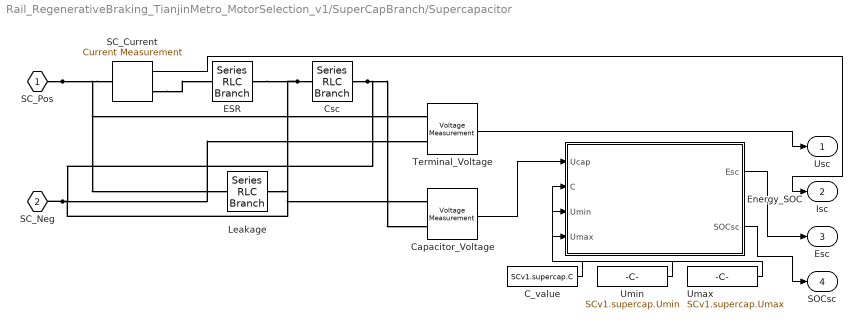
== system Rail_RegenerativeBraking_TianjinMetro_MotorSelection_v1/SuperCapBranch/Supercapacitor ==
  C_value : Constant  Value=SCv1.supercap.C
  Capacitor_Voltage : spsVoltageMeasurementLib/Voltage Measurement  PhasorSimulation=off  OutputType=Complex  PSBequivalent=0
  Csc : spsSeriesRLCBranchLib/Series RLC Branch  LConnTagsString=__new0  RConnTagsString=__new0  BranchType=C  Resistance=1  Inductance=1e-3  SetiL0=off  InitialCurrent=0  Capacitance=SCv1.supercap.C  Setx0=on  InitialVoltage=SCv1.supercap.Uinit  Measurements=None
  ESR : spsSeriesRLCBranchLib/Series RLC Branch  LConnTagsString=__new0  RConnTagsString=__new0  BranchType=R  Resistance=SCv1.supercap.ESR  Inductance=1e-3  SetiL0=off  InitialCurrent=0  Capacitance=1e-6  Setx0=off  InitialVoltage=0  Measurements=None
  Energy_SOC : MATLAB Function  TreatAsAtomicUnit=on
  Leakage : spsSeriesRLCBranchLib/Series RLC Branch  LConnTagsString=__new0  RConnTagsString=__new0  BranchType=R  Resistance=SCv1.supercap.leakage_R  Inductance=1e-3  SetiL0=off  InitialCurrent=0  Capacitance=1e-6  Setx0=off  InitialVoltage=0  Measurements=None
  SC_Current : spsCurrentMeasurementLib/Current Measurement  PhasorSimulation=off  OutputType=Complex  PSBequivalent=0
  Terminal_Voltage : spsVoltageMeasurementLib/Voltage Measurement  PhasorSimulation=off  OutputType=Complex  PSBequivalent=0
  Umax : Constant  Value=SCv1.supercap.Umax
  Umin : Constant  Value=SCv1.supercap.Umin
  SC_Pos : PMIOPort  Side=Left
  SC_Neg : PMIOPort  Port=2  Side=Left
  Usc : Outport
  Isc : Outport  Port=2
  Esc : Outport  Port=3
  SOCsc : Outport  Port=4
  wires:
  Capacitor_Voltage/1 -> Energy_SOC/1(Ucap)
  C_value/1 -> Energy_SOC/2(C)
  Umin/1 -> Energy_SOC/3(Umin)
  Umax/1 -> Energy_SOC/4(Umax)
  Terminal_Voltage/1 -> Usc/1
  SC_Current/1 -> Isc/1
  Energy_SOC/1(Esc) -> Esc/1
  Energy_SOC/2(SOCsc) -> SOCsc/1
  connections:
  SC_Current/LConn1 -- SC_Pos/RConn1 -- Leakage/LConn1 -- Terminal_Voltage/LConn1
  SC_Current/RConn1 -- ESR/LConn1
  Csc/LConn1 -- ESR/RConn1 -- Capacitor_Voltage/LConn1
  Csc/RConn1 -- Capacitor_Voltage/LConn2 -- Leakage/RConn1 -- SC_Neg/RConn1 -- Terminal_Voltage/LConn2

== system Rail_RegenerativeBraking_TianjinMetro_MotorSelection_v1/TractionBrakeSupervisor/Speed_PI_Reused ==
  note: Pierre Giroux, Gilbert Sybille
      | Power System Simulation Laboratory
      | IREQ, Hydro-Quebc
  note: Discrete PID Controller
  Error : Inport  SampleTime=Ts
  Discrete-Time Integrator : DiscreteIntegrator  InitialCondition=Init  SampleTime=Ts  LimitOutput=on  UpperSaturationLimit=UpperLimit  LowerSaturationLimit=LowerLimit  ICPrevOutput=DiscIntNeverNeededParam  ICPrevScaledInput=DiscIntNeverNeededParam
  Kp1 : Gain  Gain=Ba  SaturateOnIntegerOverflow=on  SampleTime=Ts  OutDataTypeStr=Inherit: Same as input  ParamDataTypeStr=Inherit: Same as input
  Kp4 : Gain  Gain=Kpw  SaturateOnIntegerOverflow=on  SampleTime=Ts  OutDataTypeStr=Inherit: Same as input  ParamDataTypeStr=Inherit: Same as input
  Kp5 : Gain  Gain=Kiw  SaturateOnIntegerOverflow=on  SampleTime=Ts  OutDataTypeStr=Inherit: Same as input  ParamDataTypeStr=Inherit: Same as input
  Saturation2 : Saturate  UpperLimit=UpperLimit  LowerLimit=LowerLimit  SampleTime=Ts
  Sum6 : Sum  Inputs=++-  InputSameDT=on  SaturateOnIntegerOverflow=on  SampleTime=Ts  OutDataTypeStr=Inherit: Same as first input
  Zero-Order Hold : ZeroOrderHold  SampleTime=Ts
  Out : Outport  SampleTime=Ts  InitialOutput=0
  wires:
  Kp1/1 -> Sum6/3
  Sum6/1 -> Saturation2/1
  Kp5/1 -> Discrete-Time Integrator/1
  Kp4/1 -> Zero-Order Hold/1
  Discrete-Time Integrator/1 -> Sum6/2
  Saturation2/1 -> Out/1
  Zero-Order Hold/1 -> Sum6/1
  Error/1 -> Kp4/1, Kp5/1, Kp1/1

== system Rail_RegenerativeBraking_TianjinMetro_MotorSelection_v1/TractionDrive/Anti_Park ==
  Vq : Inport
  Vd : Inport  Port=2
  Fcn : Fcn  Expr=cos(u[1])*u[2]-sin(u[1])*u[3]
  Fcn1 : Fcn  Expr=sin(u[1])*u[2]+cos(u[1])*u[3]
  Mux1 : Mux  Inputs=3
  Ualpha : Outport
  Ubeta : Outport  Port=2
  wires:
  Fcn1/1 -> Ubeta/1
  Fcn/1 -> Ualpha/1
  Mux1/1 -> Fcn/1, Fcn1/1
  Vd/1 -> Mux1/2
  Vq/1 -> Mux1/3
  [The] -> Mux1/1

== system Rail_RegenerativeBraking_TianjinMetro_MotorSelection_v1/TractionDrive/Clark ==
  A : Inport
  B : Inport  Port=2
  C : Inport  Port=3
  Mux : Mux  Inputs=3
  alpha : Fcn  Expr=(u(1)-0.5*(u(2)+u(3)))*2/3
  beta : Fcn  Expr=sqrt(3)/2*(u(2)-u(3))*2/3
  Alpha : Outport
  Beta : Outport  Port=2
  wires:
  alpha/1 -> Alpha/1
  B/1 -> Mux/2
  C/1 -> Mux/3
  A/1 -> Mux/1
  Mux/1 -> beta/1, alpha/1
  beta/1 -> Beta/1

== system Rail_RegenerativeBraking_TianjinMetro_MotorSelection_v1/TractionDrive/Mux ==
  m : Inport
  Bus Selector : BusSelector  OutputSignals=Stator current is_a (A),Stator current is_b (A),Stator current is_c (A)
  Bus Selector1 : BusSelector  OutputSignals=Rotor speed wm (rad/s),Rotor angle thetam (rad),Electromagnetic torque Te (N*m)
  Mux : Mux  Inputs=3
  Te : Outport
  The : Outport  Port=2
  Iabc : Outport  Port=3
  Wm : Outport  Port=4
  wires:
  Bus Selector1/1 -> Wm/1  "<Rotor speed wm (rad/s)>"
  Bus Selector1/2 -> The/1  "<Rotor angle thetam (rad)>"
  Bus Selector1/3 -> Te/1  "<Electromagnetic torque Te (N*m)>"
  m/1 -> Bus Selector/1, Bus Selector1/1
  Bus Selector/2 -> Mux/2  "<Stator current is_b (A)>"
  Bus Selector/3 -> Mux/3  "<Stator current is_c (A)>"
  Bus Selector/1 -> Mux/1  "<Stator current is_a (A)>"
  Mux/1 -> Iabc/1

== system Rail_RegenerativeBraking_TianjinMetro_MotorSelection_v1/TractionDrive/Plark ==
  Alpha : Inport
  Beta : Inport  Port=2
  The : Inport  Port=3
  Mux : Mux  Inputs=3
  d : Fcn  Expr=u(1)*cos(u(3))+u(2)*sin(u(3))
  q : Fcn  Expr=-u(1)*sin(u(3))+u(2)*cos(u(3))
  D : Outport
  Q : Outport  Port=2
  wires:
  d/1 -> D/1
  Beta/1 -> Mux/2
  Alpha/1 -> Mux/1
  Mux/1 -> q/1, d/1
  q/1 -> Q/1
  The/1 -> Mux/3

== system Rail_RegenerativeBraking_TianjinMetro_MotorSelection_v1/TractionDrive/SVPWM ==
  Valpha : Inport
  Vbeta : Inport  Port=2
  Udc : Inport  Port=3
  PWM : Subsystem
  Repeating Sequence : simulink/Sources/Repeating Sequence  rep_seq_t=[0 0.00005 0.0001]  rep_seq_y=[0 0.00005 0]
  Sector Caculate : Subsystem
  T1T1 Caculate : Subsystem
  Tcm Caculate : Subsystem
  Tpwm : Constant  Value=0.0001
  XYZ Caculate : Subsystem
  pulse : Outport
  wires:
  PWM/1(PWM) -> pulse/1
  Repeating Sequence/1 -> PWM/1(In)
  Vbeta/1 -> XYZ Caculate/2(Ubeta), Sector Caculate/2(Ubeta)
  T1T1 Caculate/1(T1) -> Tcm Caculate/2(T1)
  Valpha/1 -> XYZ Caculate/1(Ualpha), Sector Caculate/1(Ualpha)
  T1T1 Caculate/2(T2) -> Tcm Caculate/3(T2)
  Sector Caculate/1("N ") -> Tcm Caculate/1(N), T1T1 Caculate/1(N)
  XYZ Caculate/1(XYZ) -> T1T1 Caculate/2(XYZ)
  Tpwm/1 -> XYZ Caculate/3(Ts), Tcm Caculate/4(Tpwm), T1T1 Caculate/3(Tpwm)
  Tcm Caculate/1(Tcm1 Tcm2 Tcm3) -> PWM/2(Tcm123)
  Udc/1 -> XYZ Caculate/4(Udc)

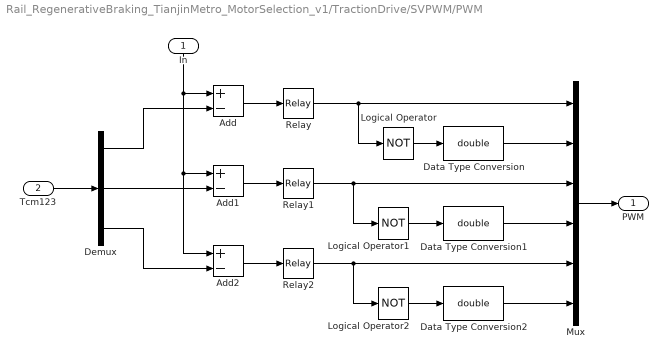
== system Rail_RegenerativeBraking_TianjinMetro_MotorSelection_v1/TractionDrive/SVPWM/PWM ==
  In : Inport
  Tcm123 : Inport  Port=2
  Add : Sum  Inputs=+-
  Add1 : Sum  Inputs=+-
  Add2 : Sum  Inputs=+-
  Data Type Conversion : DataTypeConversion  OutDataTypeStr=double  SaturateOnIntegerOverflow=off  RndMeth=Floor
  Data Type Conversion1 : DataTypeConversion  OutDataTypeStr=double  SaturateOnIntegerOverflow=off  RndMeth=Floor
  Data Type Conversion2 : DataTypeConversion  OutDataTypeStr=double  SaturateOnIntegerOverflow=off  RndMeth=Floor
  Demux : Demux  Outputs=3
  Logical Operator : Logic  Operator=NOT  AllPortsSameDT=off  OutDataTypeStr=boolean
  Logical Operator1 : Logic  Operator=NOT  AllPortsSameDT=off  OutDataTypeStr=boolean
  Logical Operator2 : Logic  Operator=NOT  AllPortsSameDT=off  OutDataTypeStr=boolean
  Mux : Mux  Inputs=6
  Relay : Relay  OffSwitchValue=-eps
  Relay1 : Relay  OffSwitchValue=-eps
  Relay2 : Relay  OffSwitchValue=-eps
  PWM : Outport
  wires:
  Demux/3 -> Add2/2
  Demux/2 -> Add1/2
  Demux/1 -> Add/2
  Relay2/1 -> Mux/5, Logical Operator2/1
  Relay1/1 -> Mux/3, Logical Operator1/1
  Relay/1 -> Logical Operator/1, Mux/1
  Mux/1 -> PWM/1
  Data Type Conversion/1 -> Mux/2
  Data Type Conversion1/1 -> Mux/4
  Data Type Conversion2/1 -> Mux/6
  Logical Operator2/1 -> Data Type Conversion2/1
  Logical Operator1/1 -> Data Type Conversion1/1
  Logical Operator/1 -> Data Type Conversion/1
  Add1/1 -> Relay1/1
  Add2/1 -> Relay2/1
  Add/1 -> Relay/1
  In/1 -> Add/1, Add2/1, Add1/1
  Tcm123/1 -> Demux/1

== system Rail_RegenerativeBraking_TianjinMetro_MotorSelection_v1/TractionDrive/SVPWM/Sector Caculate ==
  Ualpha : Inport
  Ubeta : Inport  Port=2
  B0 : Fcn  Expr=u[2]
  B1 : Fcn  Expr=u[1]*sqrt(3/4)-0.5*u[2]
  B2 : Fcn  Expr=-u[1]*sqrt(3/4)-u[2]*0.5
  Constant : Constant
  Constant1 : Constant  Value=0
  Mux : Mux  Inputs=2
  Mux1 : Mux  Inputs=3
  N : Fcn  Expr=4*u[3]+2*u[2]+u[1]
  Switch : Switch  SaturateOnIntegerOverflow=off  InputSameDT=off
  Switch1 : Switch  SaturateOnIntegerOverflow=off  InputSameDT=off
  Switch2 : Switch  SaturateOnIntegerOverflow=off  InputSameDT=off
  "N " : Outport
  wires:
  Switch2/1 -> Mux1/3
  Switch/1 -> Mux1/1
  Ualpha/1 -> Mux/1
  Ubeta/1 -> Mux/2
  Mux/1 -> B2/1, B1/1, B0/1
  B0/1 -> Switch/2
  B1/1 -> Switch1/2
  B2/1 -> Switch2/2
  Constant/1 -> Switch/1, Switch2/1, Switch1/1
  Constant1/1 -> Switch/3, Switch1/3, Switch2/3
  Switch1/1 -> Mux1/2
  Mux1/1 -> N/1
  N/1 -> "N "/1

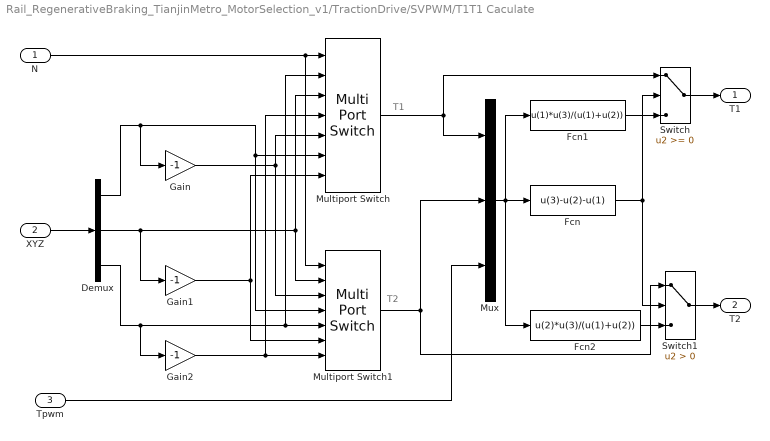
== system Rail_RegenerativeBraking_TianjinMetro_MotorSelection_v1/TractionDrive/SVPWM/T1T1 Caculate ==
  note: T1
  note: T2
  N : Inport
  XYZ : Inport  Port=2
  Tpwm : Inport  Port=3
  Demux : Demux  Outputs=3
  Fcn : Fcn  Expr=u(3)-u(2)-u(1)
  Fcn1 : Fcn  Expr=u(1)*u(3)/(u(1)+u(2))
  Fcn2 : Fcn  Expr=u(2)*u(3)/(u(1)+u(2))
  Gain : Gain  Gain=-1
  Gain1 : Gain  Gain=-1
  Gain2 : Gain  Gain=-1
  Multiport Switch : MultiPortSwitch  Inputs=6  DiagnosticForDefault=None  SaturateOnIntegerOverflow=off  InputSameDT=off
  Multiport Switch1 : MultiPortSwitch  Inputs=6  DiagnosticForDefault=None  SaturateOnIntegerOverflow=off  InputSameDT=off
  Mux : Mux  Inputs=3
  Switch : Switch  SaturateOnIntegerOverflow=off  InputSameDT=off
  Switch1 : Switch  Criteria=u2 > Threshold  SaturateOnIntegerOverflow=off  InputSameDT=off
  T1 : Outport
  T2 : Outport  Port=2
  wires:
  Tpwm/1 -> Mux/3
  XYZ/1 -> Demux/1
  Switch1/1 -> T2/1
  Switch/1 -> T1/1
  Fcn2/1 -> Switch1/3
  Fcn1/1 -> Switch/3
  Fcn/1 -> Switch/2, Switch1/2
  Mux/1 -> Fcn1/1, Fcn/1, Fcn2/1
  Multiport Switch/1 -> Switch/1, Mux/1
  Multiport Switch1/1 -> Switch1/1, Mux/2
  N/1 -> Multiport Switch/1, Multiport Switch1/1
  Demux/2 -> Multiport Switch/3, Multiport Switch1/2, Gain1/1
  Demux/3 -> Multiport Switch1/5, Multiport Switch/2, Gain2/1
  Demux/1 -> Multiport Switch/6, Multiport Switch1/4, Gain/1
  Gain/1 -> Multiport Switch1/3, Multiport Switch/5
  Gain2/1 -> Multiport Switch/4, Multiport Switch1/7
  Gain1/1 -> Multiport Switch1/6, Multiport Switch/7

== system Rail_RegenerativeBraking_TianjinMetro_MotorSelection_v1/TractionDrive/SVPWM/Tcm Caculate ==
  N : Inport
  T1 : Inport  Port=2
  T2 : Inport  Port=3
  Tpwm : Inport  Port=4
  Fcn : Fcn  Expr=(u[3]-u[1]-u[2])/4
  Fcn1 : Fcn  Expr=(u[3]+u[1]-u[2])/4
  Fcn2 : Fcn  Expr=(u[3]+u[2]+u[1])/4
  Multiport Switch : MultiPortSwitch  Inputs=6  DiagnosticForDefault=None  SaturateOnIntegerOverflow=off  InputSameDT=off
  Multiport Switch1 : MultiPortSwitch  Inputs=6  DiagnosticForDefault=None  SaturateOnIntegerOverflow=off  InputSameDT=off
  Multiport Switch2 : MultiPortSwitch  Inputs=6  DiagnosticForDefault=None  SaturateOnIntegerOverflow=off  InputSameDT=off
  Mux : Mux  Inputs=3
  Mux1 : Mux  Inputs=3
  Tcm1 Tcm2 Tcm3 : Outport
  wires:
  Mux/1 -> Fcn2/1, Fcn/1, Fcn1/1
  Tpwm/1 -> Mux/3
  T2/1 -> Mux/2
  T1/1 -> Mux/1
  Multiport Switch2/1 -> Mux1/3
  Multiport Switch1/1 -> Mux1/2
  Multiport Switch/1 -> Mux1/1
  Mux1/1 -> Tcm1 Tcm2 Tcm3/1
  Fcn/1 -> Multiport Switch/3, Multiport Switch/4, Multiport Switch1/6, Multiport Switch2/5, Multiport Switch2/7, Multiport Switch1/2
  Fcn1/1 -> Multiport Switch1/5, Multiport Switch2/3, Multiport Switch2/6, Multiport Switch1/4, Multiport Switch/7, Multiport Switch/2
  Fcn2/1 -> Multiport Switch/5, Multiport Switch/6, Multiport Switch1/3, Multiport Switch1/7, Multiport Switch2/2, Multiport Switch2/4
  N/1 -> Multiport Switch2/1, Multiport Switch1/1, Multiport Switch/1

== system Rail_RegenerativeBraking_TianjinMetro_MotorSelection_v1/TractionDrive/SVPWM/XYZ Caculate ==
  Ualpha : Inport
  Ubeta : Inport  Port=2
  Ts : Inport  Port=3
  Udc : Inport  Port=4
  Add : Sum
  Add1 : Sum  Inputs=+-
  Gain : Gain  Gain=3/2
  Gain1 : Gain  Gain=sqrt(3)
  Gain2 : Gain  Gain=sqrt(3)/2
  Math Function : Math  Operator=reciprocal  SignedPower=on
  Mux : Mux  Inputs=3
  Product{,1..3} (4 alike) : Product  RndMeth=Zero
  XYZ : Outport
  wires:
  Mux/1 -> XYZ/1
  Product1/1 -> Mux/1
  Product3/1 -> Mux/2
  Product2/1 -> Mux/3
  Ualpha/1 -> Gain/1
  Ubeta/1 -> Gain2/1, Gain1/1
  Udc/1 -> Math Function/1
  Math Function/1 -> Product/2
  Ts/1 -> Product/1
  Gain1/1 -> Product1/1
  Product/1 -> Product2/2, Product1/2, Product3/2
  Gain/1 -> Add1/2, Add/2
  Gain2/1 -> Add/1, Add1/1
  Add1/1 -> Product2/1
  Add/1 -> Product3/1

== matlab function Rail_RegenerativeBraking_TianjinMetro_MotorSelection_v1/DCBus/Power_to_Current ==
  data: Te input; omega_m input; I output; drive_units input; Vnom input; eta input; Ilimit input
function I = fcn(Te,omega_m,drive_units,Vnom,eta,Ilimit)
Pmech = Te*omega_m;
if Pmech >= 0
    Pelec = Pmech/max(eta,0.1);
else
    Pelec = Pmech*eta;
end
I = min(max((max(drive_units,1)-1)*Pelec/max(Vnom,100),-Ilimit),Ilimit);
end

== matlab function Rail_RegenerativeBraking_TianjinMetro_MotorSelection_v1/SuperCapBranch/Supercapacitor/Energy_SOC ==
  data: Ucap input; Esc output; C input; Umin input; Umax input; SOCsc output
function [Esc,SOCsc] = fcn(Ucap,C,Umin,Umax)
Esc = 0.5*C*Ucap*Ucap;
SOCsc = min(max((Ucap*Ucap-Umin*Umin)/(Umax*Umax-Umin*Umin),0),1);
end

== matlab function Rail_RegenerativeBraking_TianjinMetro_MotorSelection_v1/SuperCapBranch/BidirectionalDCDC_SC/Udc_Charge_Controller ==
  data: Udc input; Isc_cmd output; Usc input; SOCsc input; BrakeActive input; SC_Enable input; Udc_on input; Udc_target input; Udc_discharge input; SOCmax input; SOCmin input; Umax input; Umin input; Imax input; Kp input; enableDischarge input; Duty output; Mode output
function [Isc_cmd,Duty,Mode] = fcn(Udc,Usc,SOCsc,BrakeActive,SC_Enable,Udc_on,Udc_target,Udc_discharge,SOCmax,SOCmin,Umax,Umin,Imax,Kp,enableDischarge)
Isc_cmd = 0; Duty = 0; Mode = 0;
if SC_Enable > 0.5 && BrakeActive > 0.5 && Udc > Udc_on && SOCsc < SOCmax && Usc < Umax
    fsoc = min(max((SOCmax-SOCsc)/0.03,0),1);
    fvolt = min(max((Umax-Usc)/10,0),1);
    Isc_cmd = min(max(Kp*(Udc-Udc_target),0),Imax)*fsoc*fvolt;
    Duty = min(max(Usc/max(Udc,100),0.02),0.95); Mode = 1;
elseif SC_Enable > 0.5 && enableDischarge > 0.5 && BrakeActive < 0.5 && Udc < Udc_discharge && SOCsc > SOCmin && Usc > Umin
    Isc_cmd = -min(Kp*(Udc_discharge-Udc),Imax);
    Duty = min(max(1-Usc/max(Udc,100),0.02),0.95); Mode = 2;
end
end

== matlab function Rail_RegenerativeBraking_TianjinMetro_MotorSelection_v1/SuperCapBranch/BidirectionalDCDC_SC/Power_Conservation ==
  data: Isc input; Psc output; Usc input; Udc input; Mode input; etaC input; etaD input; Ibus output
function [Psc,Ibus] = fcn(Isc,Usc,Udc,Mode,etaC,etaD)
Psc = Usc*Isc;
if Mode == 1
    Ibus = Psc/(max(Udc,100)*etaC);
elseif Mode == 2
    Ibus = Psc*etaD/max(Udc,100);
else
    Ibus = 0; Psc = 0;
end
end

== matlab function Rail_RegenerativeBraking_TianjinMetro_MotorSelection_v1/EnergyAccounting/Power_Sign_Convention ==
  data: Te input; Pmotor output; omega_m input; Udc input; Idc_unit input; Psc input; Igrid input; Fmechanical input; v_train input; N input; Vsource input; Pdc output; Pregen output; Ptraction output; PscCharge output; PgridReturn output; Pmechanical output; Idc_total output; Pgrid output
function [Pmotor,Pdc,Pregen,Ptraction,PscCharge,PgridReturn,Pmechanical,Idc_total,Pgrid] = fcn(Te,omega_m,Udc,Idc_unit,Psc,Igrid,Fmechanical,v_train,N,Vsource)
Pmotor = N*Te*omega_m;
Idc_total = N*Idc_unit;
Pdc = Udc*Idc_total;
Pregen = max(-Pdc,0);
Ptraction = max(Pdc,0);
PscCharge = max(Psc,0);
Pgrid = Vsource*Igrid;
PgridReturn = max(-Pgrid,0);
Pmechanical = max(Fmechanical,0)*max(v_train,0);
end

== matlab function Rail_RegenerativeBraking_TianjinMetro_MotorSelection_v1/EnergyAccounting/Energy_Metrics ==
  data: Etraction input; Etraction_kJ output; Eregen input; Esc input; EgridReturn input; Emechanical input; Eregen_kJ output; Eregen_Wh output; Esc_kJ output; Esc_Wh output; Egrid_return_kJ output; Emechanical_kJ output; RecoveryRatio output; BalanceError_kJ output
function [Etraction_kJ,Eregen_kJ,Eregen_Wh,Esc_kJ,Esc_Wh,Egrid_return_kJ,Emechanical_kJ,RecoveryRatio,BalanceError_kJ] = fcn(Etraction,Eregen,Esc,EgridReturn,Emechanical)
Etraction_kJ=Etraction/1000; Eregen_kJ=Eregen/1000; Eregen_Wh=Eregen/3600;
Esc_kJ=Esc/1000; Esc_Wh=Esc/3600; Egrid_return_kJ=EgridReturn/1000; Emechanical_kJ=Emechanical/1000;
RecoveryRatio=Esc/max(Eregen,1);
BalanceError_kJ=(Eregen-Esc-EgridReturn)/1000;
end

== matlab function Rail_RegenerativeBraking_TianjinMetro_MotorSelection_v1/TestScenario/Speed_Profile ==
  data: t input; v_ref output; target_speed input; accel input; start_time input; brake_start input; decel input; BrakeCmd output
function [v_ref,BrakeCmd] = fcn(t,target_speed,accel,start_time,brake_start,decel)
t_reach = start_time + target_speed/max(accel,0.01);
if t < start_time
    v_ref = 0; BrakeCmd = 0;
elseif t < t_reach
    v_ref = min(accel*(t-start_time),target_speed); BrakeCmd = 0;
elseif t < brake_start
    v_ref = target_speed; BrakeCmd = 0;
else
    v_ref = max(target_speed-decel*(t-brake_start),0); BrakeCmd = 1;
end
end
